simulink library "ca_lib"  (R2018b)
settings: Solver=VariableStepAuto  StartTime=0.0  StopTime=10.0  RelTol=1e-3
undefined symbols (not defined in the file or in its folder): ca
libraries: $bdroot x1
settings Model: Creator=Ybeyer  LastModifiedBy=yannic
settings DebuggingCC: LibraryContextMissingDiagnostic=none
settings SFSimCC: SimUseLocalCustomCode=off
settings RTWCC: RTWUseLocalCustomCode=off
settings CodeAppCC: StateflowObjectComments=on

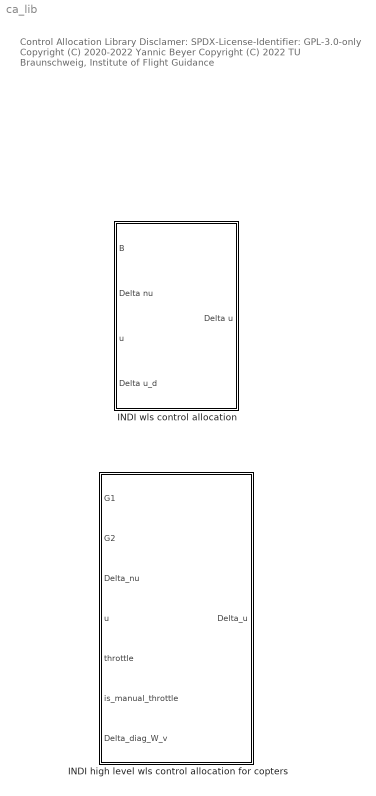
== system ca_lib ==
  note: Control Allocation Library
      |
      | Disclamer:
      | SPDX-License-Identifier: GPL-3.0-only
      |
      | Copyright (C) 2020-2022 Yannic Beyer
      | Copyright (C) 2022 TU Braunschweig, Institute of Flight Guidance
  INDI high level wls control allocation for copters : Subsystem  mask{ca=ca, is_Delta_W_v_check=on, is_W_check=off, is_iter_check=off}
      mask prompts: ca "control allocation parameters struct, see caWls_params_default"; is_Delta_W_v_check "enable online adjustment of diag W_v"; is_W_check "enable output "optimal active set" W"; is_iter_check "enable output "number of iterations" iter"
      mask init:
      | caIndiWlsHlcBlockInit(is_Delta_W_v_check,is_W_check,is_iter_check)
      | length_u = length(ca.u_min);
      mask DialogControl DescGroupVar Prompt: INDI high level control allocation
      mask DialogControl DescTextVar Prompt: It wraps the INDI control allocation block and adds some high level usability features.
      mask DialogControl Control2 Prompt: This block makes manual throttle control possible. Moreover, it not only considers the control effectiveness G1 but also the effectiveness of the control input derivative G2 [1].
      mask DialogControl Control3 Prompt: [1] Smeur, E. J., Chu, Q., & de Croon, G. C. (2016). Adaptive incremental nonlinear dynamic inversion for attitude control of micro air vehicles. Journal of Guidance, Control, and Dynamics, 39(3), 450-461.
  INDI wls control allocation : Subsystem  mask{ca=ca, is_Delta_u_d_checked=on, is_Delta_gamma_checked=off, is_Delta_W_v_checked=off, is_W_checked=off, is_iter_checked=off}
      mask prompts: ca "control allocation parameters struct, see caWls_params_default"; is_Delta_u_d_checked "enable online adjustment of u_d"; is_Delta_gamma_checked "enable online adjustment of gamma"; is_Delta_W_v_checked "enable online adjustment of diag W_v"; is_W_checked "enable output "optimal active set" W"; is_iter_checked "enable output "number of iterations" iter"
      mask init:
      | caIndiWlsBlockInit(is_Delta_u_d_checked,is_Delta_gamma_checked,is_Delta_W_v_checked,is_W_checked,is_iter_checked)
      mask DialogControl DescGroupVar Prompt: INDI control allocation
      mask DialogControl DescTextVar Prompt: Solve wls control allocation algorithm for INDI.
      mask DialogControl Control2 Prompt: For more info look inside function docu inside the block.

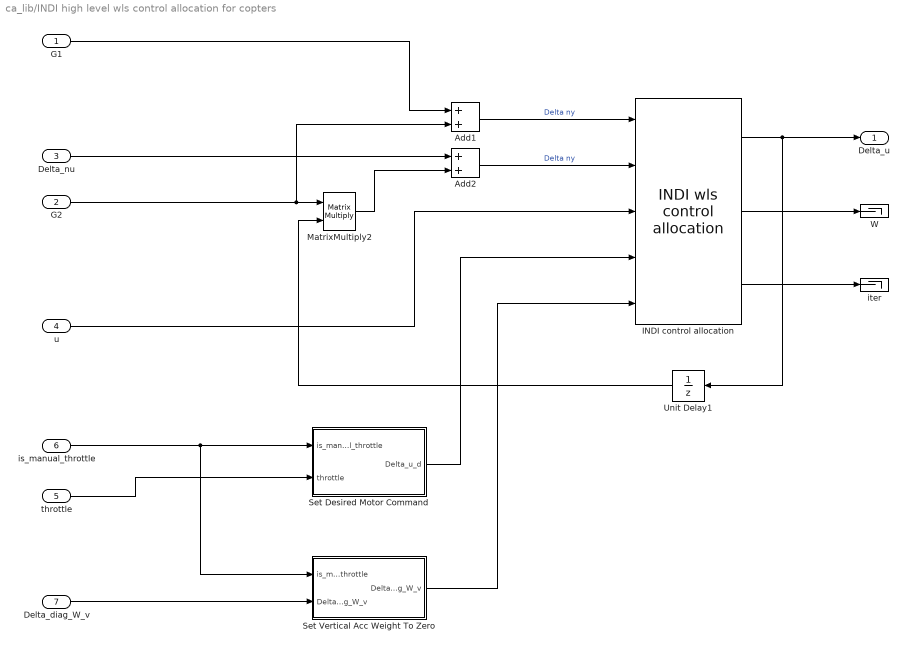
== system ca_lib/INDI high level wls control allocation for copters ==
  G1 : Inport
  G2 : Inport  Port=2
  Delta_nu : Inport  Port=3
  u : Inport  Port=4
  throttle : Inport  Port=5
  is_manual_throttle : Inport  Port=6
  Delta_diag_W_v : Inport  Port=7
  Add1 : Sum
  Add2 : Sum
  INDI control allocation : $bdroot/INDI wls control allocation  ca=ca  is_Delta_u_d_checked=on  is_Delta_gamma_checked=off  is_Delta_W_v_checked=on  is_W_checked=on  is_iter_checked=on
  MatrixMultiply2 : Product  Multiplication=Matrix(*)
  Set Desired Motor Command : MATLAB Function  TreatAsAtomicUnit=on
  Set Vertical Acc Weight To Zero : MATLAB Function  TreatAsAtomicUnit=on
  Unit Delay1 : UnitDelay  SampleTime=-1
  W : Terminator
  iter : Terminator
  Delta_u : Outport  PortDimensions=length_u
  wires:
  Delta_diag_W_v/1 -> Set Vertical Acc Weight To Zero/2("Delta_diag_W_v ")
  Set Vertical Acc Weight To Zero/1(Delta_diag_W_v) -> INDI control allocation/5
  Set Desired Motor Command/1(Delta_u_d) -> INDI control allocation/4
  is_manual_throttle/1 -> Set Vertical Acc Weight To Zero/1(is_manual_throttle), Set Desired Motor Command/1(is_manual_throttle)
  throttle/1 -> Set Desired Motor Command/2(throttle)
  G2/1 -> Add1/2, MatrixMultiply2/1
  MatrixMultiply2/1 -> Add2/2
  G1/1 -> Add1/1
  Add2/1 -> INDI control allocation/2  "Delta ny"
  u/1 -> INDI control allocation/3
  INDI control allocation/1 -> Delta_u/1, Unit Delay1/1
  Delta_nu/1 -> Add2/1
  Unit Delay1/1 -> MatrixMultiply2/2
  INDI control allocation/3 -> iter/1
  INDI control allocation/2 -> W/1
  Add1/1 -> INDI control allocation/1  "Delta ny"

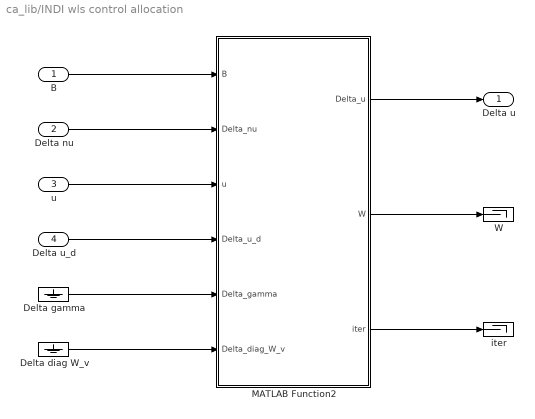
== system ca_lib/INDI wls control allocation ==
  B : Inport
  Delta nu : Inport  Port=2
  u : Inport  Port=3
  Delta u_d : Inport  Port=4
  Delta diag W_v : Ground
  Delta gamma : Ground
  MATLAB Function2 : MATLAB Function  TreatAsAtomicUnit=on
  W : Terminator
  iter : Terminator
  Delta u : Outport
  wires:
  MATLAB Function2/1(Delta_u) -> Delta u/1
  MATLAB Function2/2(W) -> W/1
  MATLAB Function2/3(iter) -> iter/1
  B/1 -> MATLAB Function2/1(B)
  Delta nu/1 -> MATLAB Function2/2(Delta_nu)
  u/1 -> MATLAB Function2/3(u)
  Delta u_d/1 -> MATLAB Function2/4(Delta_u_d)
  Delta gamma/1 -> MATLAB Function2/5(Delta_gamma)
  Delta diag W_v/1 -> MATLAB Function2/6(Delta_diag_W_v)

== matlab function ca_lib/INDI wls control allocation/MATLAB Function2 ==
  data: B input; Delta_nu input; u input; Delta_u output; Delta_u_d input; Delta_gamma input; Delta_diag_W_v input; W output; iter output; ca parameter
function [ Delta_u, W, iter ] = caIndiWls( B, Delta_nu, u, Delta_u_d, Delta_gamma, Delta_diag_W_v, ca)
[ Delta_u, W, iter ] = caIndiWls( ca, ...
    B, Delta_nu, u, Delta_u_d, Delta_gamma, Delta_diag_W_v );
end

== matlab function ca_lib/INDI high level wls control allocation for copters/Set Vertical Acc Weight To Zero ==
  data: is_manual_throttle input; Delta_diag_W_v input; Delta_diag_W_v output; ca parameter
function Delta_diag_W_v = fcn(is_manual_throttle, Delta_diag_W_v, ca)
if is_manual_throttle
    Delta_diag_W_v(4) = -ca.W_v(4,4);
    Delta_diag_W_v(1) = -ca.W_v(1,1)+1;
    Delta_diag_W_v(2) = -ca.W_v(2,2)+1;
end

== matlab function ca_lib/INDI high level wls control allocation for copters/Set Desired Motor Command ==
  data: is_manual_throttle input; throttle input; Delta_u_d output; ca parameter
function Delta_u_d = fcn(is_manual_throttle, throttle, ca)
Delta_u_d = zeros(size(ca.u_d));
if is_manual_throttle
    for i = 1:length(Delta_u_d)
        Delta_u_d(i) = max(ca.u_min(i),min(ca.u_max(i),throttle(i)))-ca.u_d(i);
    end
end
